simulink model "eml_hdl_design_patterns"  (R2026a)
settings: Solver=FixedStepDiscrete  StopTime=10
InitFcn:
  | errMsg  = ['\n\nThis model is only for demonstration purposes.\n\nPlease do not Simulate or code generate directly from this model. \n\nBefore generating code from this model please do copy the relevant blocks of interest from this model to a new model, place them in a subsystem, build a valid test bench around them.\n\nPlease refer to the example model ''eml_hdl_incrementer'' or HDLCoder documentation'];
  | error(sprintf(errMsg));
undefined symbols (not defined in the file or in its folder): C, gain_val, init_val, lower_limit, maxWordLength, thresh, upper_limit
libraries: simulink x2
(part 4 of 5)

== matlab function eml_hdl_design_patterns/Combinatorics/hierarchical_mimoparts/consts ==
  settings: sampleTime=1
  settings: fimath=|
      | fimath(...
      |     'RoundMode', 'floor',...
      |     'OverflowMode', 'wrap',...
      |     'ProductMode', 'SpecifyPrecision', ...
      |     'ProductWordLength', 32,...
      |     'ProductFractionLength', 20,...
      |     'SumMode', 'SpecifyPrecision', ...
      |     'SumWordLength', 32,...
      |     'SumFractionLength', 20,...
      |     'CastBeforeSum', true)
  data: const00 output; const01 output; const02 output; const03 output; const04 output; const05 output; const06 output; const07 output; const08 output; const09 output; const10 output; const11 output; const12 output; const13 output; const14 output; const15 output
function [const00, const01, const02, const03, ...
          const04, const05, const06, const07, ...
          const08, const09, const10, const11, ...
          const12, const13, const14, const15] = fcn

const00 = getfi([-1 -1 -1 -1], 1, 16, 10);
const01 = getfi([-1 -1 -1  1], 1, 16, 10);
const02 = getfi([-1 -1  1 -1], 1, 16, 10);
const03 = getfi([-1 -1  1  1], 1, 16, 10);

const04 = getfi([-1  1 -1 -1], 1, 16, 10);
const05 = getfi([-1  1 -1  1], 1, 16, 10);
const06 = getfi([-1  1  1 -1], 1, 16, 10);
const07 = getfi([-1  1  1  1], 1, 16, 10);

const08 = getfi([ 1 -1 -1 -1], 1, 16, 10);
const09 = getfi([ 1 -1 -1  1], 1, 16, 10);
const10 = getfi([ 1 -1  1 -1], 1, 16, 10);
const11 = getfi([ 1 -1  1  1], 1, 16, 10);

const12 = getfi([ 1 1 -1 -1], 1, 16, 10);
const13 = getfi([ 1 1 -1  1], 1, 16, 10);
const14 = getfi([ 1 1  1 -1], 1, 16, 10);
const15 = getfi([ 1 1  1  1], 1, 16, 10);

end

function myfi = getfi(input, issigned, wlen, flen)

fm = fimath(...
    'RoundMode', 'floor',...
    'OverflowMode', 'wrap',...
    'ProductMode', 'SpecifyPrecision', ...
    'ProductWordLength', 32,...
    'ProductFractionLength', 20,...
    'SumMode', 'SpecifyPrecision', ...
    'SumWordLength', 32,...
    'SumFractionLength', 20,...    
    'CastBeforeSum', true);

myfi = fi(input, issigned, wlen, flen, 'fimath', fm);

end

== matlab function eml_hdl_design_patterns/Combinatorics/hierarchical_mimoparts/distance ==
  settings: sampleTime=1
  settings: fimath=|
      | fimath(...
      |     'RoundMode', 'floor',...
      |     'OverflowMode', 'wrap',...
      |     'ProductMode', 'SpecifyPrecision', ...
      |     'ProductWordLength', 32,...
      |     'ProductFractionLength', 20,...
      |     'SumMode', 'SpecifyPrecision', ...
      |     'SumWordLength', 32,...
      |     'SumFractionLength', 20,...
      |     'CastBeforeSum', true)
  data: mpy00 input; mpy01 input; mpy02 input; mpy03 input; mpy04 input; mpy05 input; mpy06 input; mpy07 input; mpy08 input; mpy09 input; mpy10 input; mpy11 input; mpy12 input; mpy13 input; mpy14 input; mpy15 input; y_nums input fixdt(1,32,20) size=[1 4]; vec output
function vec = fcn(mpy00, mpy01, mpy02, mpy03, ...
          mpy04, mpy05, mpy06, mpy07, ...
          mpy08, mpy09, mpy10, mpy11, ...
          mpy12, mpy13, mpy14, mpy15, y_nums)

dout00 = distance(y_nums, mpy00);
dout01 = distance(y_nums, mpy01);
dout02 = distance(y_nums, mpy02);
dout03 = distance(y_nums, mpy03);

dout04 = distance(y_nums, mpy04);
dout05 = distance(y_nums, mpy05);
dout06 = distance(y_nums, mpy06);
dout07 = distance(y_nums, mpy07);

dout08 = distance(y_nums, mpy08);
dout09 = distance(y_nums, mpy09);
dout10 = distance(y_nums, mpy10);
dout11 = distance(y_nums, mpy11);

dout12 = distance(y_nums, mpy12);
dout13 = distance(y_nums, mpy13);
dout14 = distance(y_nums, mpy14);
dout15 = distance(y_nums, mpy15);

vec = [dout00, dout01, dout02, dout03, ...
               dout04, dout05, dout06, dout07, ...
               dout08, dout09, dout10, dout11, ...
               dout12, dout13, dout14, dout15];
           
end


function dout = distance(in1, in2)

sub_t1 = getfi(in1-in2, 1, 32, 20);
abs_t2 = getfi(abs(sub_t1), 1, 32, 20);
soe_t3 = getfi(sum(abs_t2), 1, 32, 20);

dout = soe_t3;

end




function myfi = getfi(input, issigned, wlen, flen)

fm = fimath(...
    'RoundMode', 'floor',...
    'OverflowMode', 'wrap',...
    'ProductMode', 'SpecifyPrecision', ...
    'ProductWordLength', 32,...
    'ProductFractionLength', 20,...
    'SumMode', 'SpecifyPrecision', ...
    'SumWordLength', 32,...
    'SumFractionLength', 20,...    
    'CastBeforeSum', true);

myfi = fi(input, issigned, wlen, flen, 'fimath', fm);

end

== matlab function eml_hdl_design_patterns/Combinatorics/hierarchical_mimoparts/multiply ==
  settings: sampleTime=1
  settings: fimath=|
      | fimath(...
      |     'RoundMode', 'floor',...
      |     'OverflowMode', 'wrap',...
      |     'ProductMode', 'SpecifyPrecision', ...
      |     'ProductWordLength', 32,...
      |     'ProductFractionLength', 20,...
      |     'SumMode', 'SpecifyPrecision', ...
      |     'SumWordLength', 32,...
      |     'SumFractionLength', 20,...
      |     'CastBeforeSum', true)
  data: const00 input; const01 input; const02 input; const03 input; const04 input; const05 input; const06 input; const07 input; const08 input; const09 input; const10 input; const11 input; const12 input; const13 input; const14 input; const15 input; mpy00 output; channel_matrix input fixdt(1,16,10) size=16; mpy01 output; mpy02 output; mpy03 output; mpy04 output; mpy05 output; mpy06 output; mpy07 output; mpy08 output; mpy09 output; mpy10 output; mpy11 output; mpy12 output; mpy13 output; mpy14 output; mpy15 output
function  [mpy00, mpy01, mpy02, mpy03, ...
          mpy04, mpy05, mpy06, mpy07, ...
          mpy08, mpy09, mpy10, mpy11, ...
          mpy12, mpy13, mpy14, mpy15] ...
          = fcn (const00, const01, const02, const03, ...
          const04, const05, const06, const07, ...
          const08, const09, const10, const11, ...
          const12, const13, const14, const15, ...
          channel_matrix)

mpy00 = matrix_product(const00, channel_matrix);
mpy01 = matrix_product(const01, channel_matrix);
mpy02 = matrix_product(const02, channel_matrix);
mpy03 = matrix_product(const03, channel_matrix);
  
mpy04 = matrix_product(const04, channel_matrix);
mpy05 = matrix_product(const05, channel_matrix);
mpy06 = matrix_product(const06, channel_matrix);
mpy07 = matrix_product(const07, channel_matrix);
  
mpy08 = matrix_product(const08, channel_matrix);
mpy09 = matrix_product(const09, channel_matrix);
mpy10 = matrix_product(const10, channel_matrix);
mpy11 = matrix_product(const11, channel_matrix);
  
mpy12 = matrix_product(const12, channel_matrix);
mpy13 = matrix_product(const13, channel_matrix);
mpy14 = matrix_product(const14, channel_matrix);
mpy15 = matrix_product(const15, channel_matrix);

end

function out = matrix_product(in1, in2)

const = in1';

sel1 = in2(1:4);
sel2 = in2(5:8);
sel3 = in2(9:12);
sel4 = in2(13:16);

mpy1 = get_mpy_fi(sel1 .* const, 1, 32, 20);
mpy2 = get_mpy_fi(sel2 .* const, 1, 32, 20);
mpy3 = get_mpy_fi(sel3 .* const, 1, 32, 20);
mpy4 = get_mpy_fi(sel4 .* const, 1, 32, 20);

soe1 = get_sum_fi(sum(mpy1), 1, 32, 20);
soe2 = get_sum_fi(sum(mpy2), 1, 32, 20);
soe3 = get_sum_fi(sum(mpy3), 1, 32, 20);
soe4 = get_sum_fi(sum(mpy4), 1, 32, 20);

out = [soe1, soe2, soe3, soe4];
end



function myfi = get_mpy_fi(input, issigned, wlen, flen)
% round to zero
fm = fimath(...
    'RoundMode', 'fix',... 
    'OverflowMode', 'wrap',...
    'ProductMode', 'SpecifyPrecision', ...
    'ProductWordLength', 32,...
    'ProductFractionLength', 20,...
    'SumMode', 'SpecifyPrecision', ...
    'SumWordLength', 32,...
    'SumFractionLength', 20,...    
    'CastBeforeSum', true);

myfi = fi(input, issigned, wlen, flen, 'fimath', fm);

end



function myfi = get_sum_fi(input, issigned, wlen, flen)
% drop round bits
fm = fimath(...
    'RoundMode', 'floor',... 
    'OverflowMode', 'wrap',...
    'ProductMode', 'SpecifyPrecision', ...
    'ProductWordLength', 32,...
    'ProductFractionLength', 20,...
    'SumMode', 'SpecifyPrecision', ...
    'SumWordLength', 32,...
    'SumFractionLength', 20,...    
    'CastBeforeSum', true);

myfi = fi(input, issigned, wlen, flen, 'fimath', fm);

end

== matlab function eml_hdl_design_patterns/Adders/signed_adder ==
  settings: fimath=|
      | fimath(...
      | 'RoundMode', 'floor',...
      | 'OverflowMode', 'wrap',...
      | 'ProductMode', 'FullPrecision', 'ProductWordLength', 32,...
      | 'SumMode', 'FullPrecision', 'SumWordLength', 32,...
      | 'CastBeforeSum', true)
  data: a input fixdt(1,3,0); sum output; b input fixdt(1,3,0)
function sum  = fcn(a, b)

% check default fimath settings on the block
% that define the following addition semantics

sum = a + b;

== matlab function eml_hdl_design_patterns/Combinatorics/hierarchical_mimoparts/tree_min ==
  settings: sampleTime=1
  settings: fimath=|
      | fimath(...
      |     'RoundMode', 'floor',...
      |     'OverflowMode', 'wrap',...
      |     'ProductMode', 'SpecifyPrecision', ...
      |     'ProductWordLength', 32,...
      |     'ProductFractionLength', 20,...
      |     'SumMode', 'SpecifyPrecision', ...
      |     'SumWordLength', 32,...
      |     'SumFractionLength', 20,...
      |     'CastBeforeSum', true)
  data: inVec input fixdt(1,32,20) size=[1 16]; idx output
function idx   = fcn(inVec)
%--------------------------------------------------------------------------
% Tree implementation min function for vector input of length 64
%--------------------------------------------------------------------------
[minimum, idx] = tree_min(inVec);
            
end

function [minval, idx] = tree_min(invec)

% initialize outputs

% first level of comparison
inidx = uint8(1:16);
[lvlonemin, lvloneidx] = vector_min(invec, inidx);

% second level of comparison
[lvltwomin, lvltwoidx] = vector_min(lvlonemin, lvloneidx);

% third level of comparison
[lvlthreemin, lvlthreeidx] = vector_min(lvltwomin, lvltwoidx);

% final comparison
[minval, idx] = vector_min(lvlthreemin, lvlthreeidx);

end

% Minimum subfuction for tree implementation
function [minvec, idxvec] = vector_min(invec, inidx)
    
lengthminvec = uint8(length(invec)/2);
%lengthminvec = uint8(bitshift(invec, -1));
minvec = getfi(zeros(lengthminvec, 1), 1, 12, 6);
idxvec = uint8(zeros(lengthminvec, 1));

for i=1:lengthminvec
    % get two consecutive values
    idx2 = int8(i)+int8(i); %i*2
    idx1 = int8(idx2) - int8(1); %i*2-1
    % get elements
    val1 = invec(idx1);
    val2 = invec(idx2);
    % compare them and select minimum
    if le(val1, val2)
        minvec(i) = val1;
        idxvec(i) = inidx(idx1);
    else
        minvec(i) = val2;
        idxvec(i) = inidx(idx2);
    end
end

end


function myfi = getfi(input, issigned, wlen, flen)

fm = fimath(...
    'RoundMode', 'floor',... 
    'OverflowMode', 'wrap',...
    'ProductMode', 'SpecifyPrecision', ...
    'ProductWordLength', 32,...
    'ProductFractionLength', 20,...
    'SumMode', 'SpecifyPrecision', ...
    'SumWordLength', 32,...
    'SumFractionLength', 20,...    
    'CastBeforeSum', true);

myfi = fi(input, issigned, wlen, flen, 'fimath', fm);

end

== matlab function eml_hdl_design_patterns/Combinatorics/monolithic_mimoparts ==
  settings: fimath=|
      | fimath(...
      |     'RoundMode', 'floor',...
      |     'OverflowMode', 'wrap',...
      |     'ProductMode', 'SpecifyPrecision', ...
      |     'ProductWordLength', 32,...
      |     'ProductFractionLength', 20,...
      |     'SumMode', 'SpecifyPrecision', ...
      |     'SumWordLength', 32,...
      |     'SumFractionLength', 20,...
      |     'CastBeforeSum', true)
  data: y_nums input fixdt(1,32,20) size=[1 4]; idx output; channel_matrix input fixdt(1,16,10) size=16
function idx = fcn(y_nums, channel_matrix)

% This function illustrates some of the key pieces of a MIMO decoder, but
% is meant only for educational value at this time.
% 
% Key MATLAB code features used in this example:
% 
% 1. Creating vector constants
% 2. Using 'SpecifyPrecision' option in fimath
% 3. Indexing of vector operands
% 4. Transpose operations
% 5. Elementwise product operations
% 6. Sum of elements operation using sum input
% 7. Tree min function implementation
% 8. Vector ports
%

const00 = getfi([-1 -1 -1 -1], 1, 16, 10);
const01 = getfi([-1 -1 -1  1], 1, 16, 10);
const02 = getfi([-1 -1  1 -1], 1, 16, 10);
const03 = getfi([-1 -1  1  1], 1, 16, 10);

const04 = getfi([-1  1 -1 -1], 1, 16, 10);
const05 = getfi([-1  1 -1  1], 1, 16, 10);
const06 = getfi([-1  1  1 -1], 1, 16, 10);
const07 = getfi([-1  1  1  1], 1, 16, 10);

const08 = getfi([ 1 -1 -1 -1], 1, 16, 10);
const09 = getfi([ 1 -1 -1  1], 1, 16, 10);
const10 = getfi([ 1 -1  1 -1], 1, 16, 10);
const11 = getfi([ 1 -1  1  1], 1, 16, 10);

const12 = getfi([ 1 1 -1 -1], 1, 16, 10);
const13 = getfi([ 1 1 -1  1], 1, 16, 10);
const14 = getfi([ 1 1  1 -1], 1, 16, 10);
const15 = getfi([ 1 1  1  1], 1, 16, 10);

mpy00 = matrix_product(const00, channel_matrix);
mpy01 = matrix_product(const01, channel_matrix);
mpy02 = matrix_product(const02, channel_matrix);
mpy03 = matrix_product(const03, channel_matrix);
  
mpy04 = matrix_product(const04, channel_matrix);
mpy05 = matrix_product(const05, channel_matrix);
mpy06 = matrix_product(const06, channel_matrix);
mpy07 = matrix_product(const07, channel_matrix);
  
mpy08 = matrix_product(const08, channel_matrix);
mpy09 = matrix_product(const09, channel_matrix);
mpy10 = matrix_product(const10, channel_matrix);
mpy11 = matrix_product(const11, channel_matrix);
  
mpy12 = matrix_product(const12, channel_matrix);
mpy13 = matrix_product(const13, channel_matrix);
mpy14 = matrix_product(const14, channel_matrix);
mpy15 = matrix_product(const15, channel_matrix);

dout00 = distance(y_nums, mpy00);
dout01 = distance(y_nums, mpy01);
dout02 = distance(y_nums, mpy02);
dout03 = distance(y_nums, mpy03);

dout04 = distance(y_nums, mpy04);
dout05 = distance(y_nums, mpy05);
dout06 = distance(y_nums, mpy06);
dout07 = distance(y_nums, mpy07);

dout08 = distance(y_nums, mpy08);
dout09 = distance(y_nums, mpy09);
dout10 = distance(y_nums, mpy10);
dout11 = distance(y_nums, mpy11);

dout12 = distance(y_nums, mpy12);
dout13 = distance(y_nums, mpy13);
dout14 = distance(y_nums, mpy14);
dout15 = distance(y_nums, mpy15);

idx = TreeMin([dout00, dout01, dout02, dout03, ...
               dout04, dout05, dout06, dout07, ...
               dout08, dout09, dout10, dout11, ...
               dout12, dout13, dout14, dout15]);
           
end

function out = matrix_product(in1, in2)

sel1 = in2(1:4);
sel2 = in2(5:8);
sel3 = in2(9:12);
sel4 = in2(13:16);

% mpy1 = getfi(sel1*in1, 1, 32, 20);
% mpy2 = getfi(sel2*in1, 1, 32, 20);
% mpy3 = getfi(sel3*in1, 1, 32, 20);
% mpy4 = getfi(sel4*in1, 1, 32, 20);

mpy1 = getfi(sel1 .* in1', 1, 32, 20);
mpy2 = getfi(sel2 .* in1', 1, 32, 20);
mpy3 = getfi(sel3 .* in1', 1, 32, 20);
mpy4 = getfi(sel4 .* in1', 1, 32, 20);

soe1 = getfi(sum(mpy1), 1, 32, 20);
soe2 = getfi(sum(mpy2), 1, 32, 20);
soe3 = getfi(sum(mpy3), 1, 32, 20);
soe4 = getfi(sum(mpy4), 1, 32, 20);

out = [soe1, soe2, soe3, soe4];

end


function dout = distance(in1, in2)

sub_t1 = getfi(in1-in2, 1, 32, 20);
abs_t2 = getfi(abs(sub_t1), 1, 32, 20);
soe_t3 = getfi(sum(abs_t2), 1, 32, 20);

dout = soe_t3;

end


function [idx, minimum]  = TreeMin(nsm)
%--------------------------------------------------------------------------
% Tree implementation min function for vector input of length 64
%--------------------------------------------------------------------------
[minimum, idx] = tree_min(nsm);
            
end

function [minval, idx] = tree_min(invec)

% initialize outputs
% minval = getfi(0, 1, 12, 6);
% idx = 0;

% first level of comparison
inidx = uint8(1:16);
[lvlonemin, lvloneidx] = vector_min(invec, inidx);

% second level of comparison
[lvltwomin, lvltwoidx] = vector_min(lvlonemin, lvloneidx);

% third level of comparison
[lvlthreemin, lvlthreeidx] = vector_min(lvltwomin, lvltwoidx);

% final comparison
[minval, idx] = vector_min(lvlthreemin, lvlthreeidx);


end

% Minimum subfuction for tree implementation
function [minvec, idxvec] = vector_min(invec, inidx)
    
lengthminvec = length(invec)/2;
%lengthminvec = uint8(bitshift(invec, -1));
minvec = getfi(zeros(lengthminvec, 1), 1, 12, 6);
idxvec = uint8(zeros(lengthminvec, 1));

for i=1:lengthminvec
    % get two consecutive values
    idx2 = int8(i)+int8(i); %i*2
    idx1 = int8(idx2) - int8(1); %i*2-1
    % get elements
    val1 = invec(idx1);
    val2 = invec(idx2);
    % compare them and select minimum
    if le(val1, val2)
        minvec(i) = val1;
        idxvec(i) = inidx(idx1);
    else
        minvec(i) = val2;
        idxvec(i) = inidx(idx2);
    end
end

end


function myfi = getfi(input, issigned, wlen, flen)

fm = fimath(...
    'RoundMode', 'floor',... 
    'OverflowMode', 'wrap',...
    'ProductMode', 'SpecifyPrecision', ...
    'ProductWordLength', 32,...
    'ProductFractionLength', 20,...
    'SumMode', 'SpecifyPrecision', ...
    'SumWordLength', 32,...
    'SumFractionLength', 20,...    
    'CastBeforeSum', true);

myfi = fi(input, issigned, wlen, flen, 'fimath', fm);

end

== matlab function eml_hdl_design_patterns/Complex/Complex Integer Delay ==
  settings: fimath=|
      | fimath(...
      | 'RoundMode', 'floor',...
      | 'OverflowMode', 'wrap',...
      | 'ProductMode', 'FullPrecision', 'ProductWordLength', 32,...
      | 'SumMode', 'FullPrecision', 'SumWordLength', 32,...
      | 'CastBeforeSum', true)
  data: u input; y output
function y = fcn(u)

% The Integer Delay block delays its input by N sample periods. 
% The block accepts one input and generates one output, both of which
% can be scalar or vector. If the input is a vector, all elements of the 
% vector are delayed by the same sample period.

% In this example N is hardwired as 4; This function behaves as Integer 
% delay block and delays inputs by 4 sample hits.

persistent u_d;
if isempty(u_d)
    u_d = fi(complex(zeros(1,4)), numerictype(u), fimath(u));
end

y = u_d(4);

u_d = [u, u_d(1), u_d(2), u_d(3)];

== matlab function eml_hdl_design_patterns/Register Files/dualport_regfile ==
  settings: fimath=|
      | fimath(...
      | 'RoundMode', 'floor',...
      | 'OverflowMode', 'wrap',...
      | 'ProductMode', 'FullPrecision', 'ProductWordLength', 32,...
      | 'SumMode', 'FullPrecision', 'SumWordLength', 32,...
      | 'CastBeforeSum', true)
  data: writedata input int8; readdata output; writeaddr input uint8; written input boolean; readaddr input uint8
function readdata = fcn(writedata, writeaddr, written, readaddr)

% Synchronous register file in eML

% this generates a "register-file" and 
% does not help infer a true RAM in synthesis

% nonetheless, they are very useful for simulation and 
% can be replaced at synthesis time with code that 
% does infer a RAM or a black-box RAM.


persistent reg_file;
if isempty(reg_file)
    reg_file = fi(zeros(1, 64), 0, 8, 0);
end

trf = reg_file;
trf(writeaddr) = writedata;

% decide new reg file based on written flag
if (written)
    new_rf = trf;
else
    new_rf = reg_file;
end

% read data
readdata = reg_file(readaddr);

% update reg file
reg_file = new_rf;

== matlab function eml_hdl_design_patterns/Register Files/triport_regfile ==
  settings: fimath=|
      | fimath(...
      | 'RoundMode', 'floor',...
      | 'OverflowMode', 'wrap',...
      | 'ProductMode', 'FullPrecision', 'ProductWordLength', 32,...
      | 'SumMode', 'FullPrecision', 'SumWordLength', 32,...
      | 'CastBeforeSum', true)
  data: writedata input int8; readdata_a output; writeaddr input uint8; written input boolean; readaddr_a input uint8; readaddr_b input uint8; readdata_b output
function [readdata_a, readdata_b]= fcn(writedata, writeaddr, written, readaddr_a, readaddr_b)

% Synchronous Dual Port register file in eML

% this generates a "register-file" and 
% does not help infer a true RAM in synthesis
% Nonetheless, they are very useful for simulation and 
% can be replaced at synthesis time with code that 
% does infer a RAM or a black-box RAM.


persistent reg_file;
if isempty(reg_file)
    reg_file = fi(zeros(1, 64), 0, 8, 0);
end

trf = reg_file;
trf(writeaddr) = writedata;

% decide new reg file based on written flag
if (written)
    new_rf = trf;
else
    new_rf = reg_file;
end

% read data portA
readdata_a = reg_file(readaddr_a);

% read data portB
readdata_b = reg_file(readaddr_b);

% update reg file
reg_file = new_rf;

== matlab function eml_hdl_design_patterns/ShiftAdd Algs/cordic/InitValues/Init ==
  settings: fimath=|
      | fimath(...
      | 'RoundMode', 'floor',...
      | 'OverflowMode', 'wrap',...
      | 'ProductMode', 'FullPrecision', 'ProductWordLength', 32,...
      | 'SumMode', 'FullPrecision', 'SumWordLength', 32,...
      | 'CastBeforeSum', true)
  data: x0 output fixdt(1,24,8); y0 output fixdt(1,24,8); h_mode output boolean; r0 output fixdt(1,24,8); rot_mode output uint8; lut_values output fixdt(1,16,8) size=[1 8]; p_or_rate output uint8; cordic_gain output fixdt(1,24,23); angle_gain output fixdt(1,24,22)
function [x0, y0, ...    
    h_mode,...
    r0, rot_mode, ...    
    lut_values, ...
    p_or_rate, ...
    cordic_gain, ...
    angle_gain] = INIT

% from mask input
p_or_rate = uint8(8);

x0 = getfi(1); 
y0 = getfi(0);

r0 = getfi(0);

% hyperbolic mode
h_mode = false;

% rotation mode
rot_mode = uint8(2); 

%cg = 1/get_cordic_gain(8, 'Circular');
%cordic_gain = fi(cg, 1, 24, 23);
cordic_gain = fi(0.607259154319763, 1, 24, 23);

angle_gain = fi(1, 1, 24, 22);

%sincos_val = (atan([1, 1/2, 1/4, 1/8, 1/16, 1/32, 1/64, 1/128]))*180/pi;
%lut_values = fi(sincos_val, 1, 16, 8);

lut_values = fi([45, 26.56640625, 14.03515625, 7.125, 3.578125, 1.7890625, 0.89453125, 0.44921875], 1, 16, 8);


function fival = getfi(val)

nt = numerictype(1, 24, 8);

fm = fimath(...
    'RoundMode', 'floor',...
    'OverflowMode', 'wrap',...
    'ProductMode', 'FullPrecision', 'ProductWordLength', 32,...
    'SumMode', 'FullPrecision', 'SumWordLength', 32,...
    'CastBeforeSum', true);

fival = fi(val, nt, fm);

== matlab function eml_hdl_design_patterns/ShiftAdd Algs/cordic/cordic_core/Q Correction ==
  settings: fimath=|
      | fimath(...
      | 'RoundMode', 'floor',...
      | 'OverflowMode', 'wrap',...
      | 'ProductMode', 'FullPrecision', 'ProductWordLength', 32,...
      | 'SumMode', 'FullPrecision', 'SumWordLength', 32,...
      | 'CastBeforeSum', true)
  data: theta input fixdt(1,24,8); left_quad output; angle output
function [left_quad, angle] = Q_Correction(theta)

angle = theta;
left_quad = angle <= 270 && angle >= 90;

if left_quad
    angle = getfi(angle - getfi(180));
end


function fival = getfi(val)

nt = numerictype(1, 24, 8);

fm = fimath(...
    'RoundMode', 'floor',...
    'OverflowMode', 'wrap',...
    'ProductMode', 'FullPrecision', 'ProductWordLength', 32,...
    'SumMode', 'FullPrecision', 'SumWordLength', 32,...
    'CastBeforeSum', true);

fival = fi(val, nt, fm);

== matlab function eml_hdl_design_patterns/Counters/gray_counter ==
  settings: sampleTime=.1
  settings: fimath=|
      | fimath(...
      | 'RoundMode', 'floor',...
      | 'OverflowMode', 'wrap',...
      | 'ProductMode', 'FullPrecision', 'ProductWordLength', 32,...
      | 'SumMode', 'FullPrecision', 'SumWordLength', 32,...
      | 'CastBeforeSum', true)
  data: clear input boolean; count output fixdt(0,4,0) size=1
function count = fcn(clear)

% A gray counter is a binary counter with the following conversion logic:

% 1. the first gray bit (msb) is same as first binary bit
% 2. the second gray bit is determined by xoring the second binary with the first binary bit and so on;
%    that is each pair of adjacent bits are xor'ed to get the next gray bit.
%
% This counter is configured to rollover.  Set result_fm to 'saturate'
% if roll over is not desirable.

result_nt = numerictype(0,4,0);
result_fm = fimath('OverflowMode', 'wrap', 'RoundMode', 'floor');

persistent bin_count;
if isempty(bin_count)
    bin_count = fi(0, result_nt, result_fm);
end

persistent gray_count;
if isempty(gray_count)
    gray_count = fi(0, result_nt, result_fm); %#ok<NASGU>
end

count = gray_count;

if clear
    bin_count =  fi(0, result_nt, result_fm);
    gray_count =  fi(0, result_nt, result_fm);
else
    inc = bin_count + fi(1, result_nt, result_fm);
    bin_count = fi(inc, result_nt, result_fm);

    gray_count = bitshift(bin_count, -1);
    gray_count = bitxor( gray_count, bin_count );
end

== matlab function eml_hdl_design_patterns/Complex/Complex Tap Delay ==
  settings: fimath=|
      | fimath(...
      | 'RoundMode', 'floor',...
      | 'OverflowMode', 'wrap',...
      | 'ProductMode', 'FullPrecision', 'ProductWordLength', 32,...
      | 'SumMode', 'FullPrecision', 'SumWordLength', 32,...
      | 'CastBeforeSum', true)
  data: u input; d1 output; d2 output; d3 output; d4 output
function [d1, d2, d3, d4] = fcn(u)
%The Tapped Delay function delays its input by the specified number 
% of sample periods, and outputs all the delayed versions.

% In this example N is hardwired to 4.

persistent u_d;
if isempty(u_d)
    u_d = fi(complex(zeros(1,4)), numerictype(u), fimath(u));
end

d1 = u_d(1);
d2 = u_d(2);
d3 = u_d(3);
d4 = u_d(4);

u_d = [u_d(1), u_d(2), u_d(3), u];

== matlab function eml_hdl_design_patterns/Word Twiddlers/signal_distance ==
  settings: fimath=|
      | fimath(...
      | 'RoundMode', 'floor',...
      | 'OverflowMode', 'wrap',...
      | 'ProductMode', 'FullPrecision', 'ProductWordLength', 32,...
      | 'SumMode', 'FullPrecision', 'SumWordLength', 32,...
      | 'CastBeforeSum', true)
  data: u input fixdt(0,5,0); y output; v input fixdt(0,5,0)
function y = fcn(u, v)

% get all bits of u
t1 = bitget(u, int8(5:-1:1));

% get all bits of v in reverse order
t2 = bitget(v, int8(1:1:5));

% xor the bits
t3 = xor(t1, t2);

% find number of bits that are equal to 1

t = uint8(t3);
y = uint8(0);
for i=uint8(1:5)
    y = y+t(i);
end

== matlab function eml_hdl_design_patterns/ShiftAdd Algs/cordic/cordic_core/controller ==
  settings: updateMethod=DISCRETE  sampleTime=1/8
  settings: fimath=|
      | fimath(...
      | 'RoundMode', 'floor',...
      | 'OverflowMode', 'wrap',...
      | 'ProductMode', 'FullPrecision', 'ProductWordLength', 32,...
      | 'SumMode', 'FullPrecision', 'SumWordLength', 32,...
      | 'CastBeforeSum', true)
  data: ctrl output; address output; d_valid output; rate input
function [ctrl,address,d_valid] = controller(rate)

persistent count;
if isempty(count)
    count = uint8(1);
end

% output address
address = count;

% update count value
count = get_en_ctr_val(rate);

% send control signals based on current count value
ctrl = (count == 1);
d_valid = (count == 8);



function count = get_en_ctr_val(rate)

persistent count_val;
if isempty(count_val)
    count_val = uint8(1);
end

% output count
count = count_val;

% update count
if count >= rate
    next_cnt_val = uint8(1);
else
    next_cnt_val = uint8(count+1);
end


count_val = uint8(next_cnt_val);

== matlab function eml_hdl_design_patterns/ShiftAdd Algs/cordic/cordic_core/cordic_rotator/get_sign ==
  settings: fimath=|
      | fimath(...
      | 'RoundMode', 'floor',...
      | 'OverflowMode', 'wrap',...
      | 'ProductMode', 'FullPrecision', 'ProductWordLength', 32,...
      | 'SumMode', 'FullPrecision', 'SumWordLength', 32,...
      | 'CastBeforeSum', true)
  data: y input; x input; z input; r0 input; sign output boolean; r_mode input
function sign = get_sign(y, x, z, r0, r_mode)

sign = false;

switch (r_mode)
    case 0
        sign = x <= r0;
    case 1
        sign = y  <= r0;
    case 2
        sign = z >= r0;
end

== matlab function eml_hdl_design_patterns/ShiftAdd Algs/cordic/cordic_core/cordic_rotator/x_comp ==
  settings: fimath=|
      | fimath(...
      | 'RoundMode', 'floor',...
      | 'OverflowMode', 'wrap',...
      | 'ProductMode', 'FullPrecision', 'ProductWordLength', 32,...
      | 'SumMode', 'FullPrecision', 'SumWordLength', 32,...
      | 'CastBeforeSum', true)
  data: y input fixdt(1,24,8) size=1; next_x output fixdt(1,24,8) size=1; x0 input fixdt(1,24,8) size=1; h_mode input boolean size=1; ctrl input boolean size=1; addr input uint8 size=1; sign input boolean; store_x output fixdt(1,24,8); reg_x input fixdt(1,24,8)
function [next_x, store_x]   = x_comp(y, x0, h_mode, ctrl, addr, sign, reg_x)

y = bitshift(y, -int8(addr-1));

if h_mode    
    new_sign = sign;
else
    new_sign = ~sign;
end

next_x = z_accumulator(new_sign, reg_x, y);

% update delay line
if (ctrl)
    store_x = x0;
else
    store_x = next_x;
end


function acc = z_accumulator(add, x, y)

if (add)
    acc = getfi(x+y);
else
    acc = getfi(x-y);
end


function fival = getfi(val)

nt = numerictype(1, 24, 8);
fm = fimath(...
    'RoundMode', 'floor',...
    'OverflowMode', 'wrap',...
    'ProductMode', 'FullPrecision', 'ProductWordLength', 32,...
    'SumMode', 'FullPrecision', 'SumWordLength', 32,...
    'CastBeforeSum', true);

fival = fi(val, nt, fm);

== matlab function eml_hdl_design_patterns/ShiftAdd Algs/cordic/cordic_core/cordic_rotator/y_comp ==
  settings: fimath=|
      | fimath(...
      | 'RoundMode', 'floor',...
      | 'OverflowMode', 'wrap',...
      | 'ProductMode', 'FullPrecision', 'ProductWordLength', 32,...
      | 'SumMode', 'FullPrecision', 'SumWordLength', 32,...
      | 'CastBeforeSum', true)
  data: next_y output fixdt(1,24,8); x input fixdt(1,24,8); y0 input fixdt(1,24,8); ctrl input boolean; addr input uint8; sign input boolean; store_y output fixdt(1,24,8); reg_y input fixdt(1,24,8)
function [next_y, store_y]  = y_comp(x, y0, ctrl, addr, sign, reg_y)

x = bitshift(x, -int8(addr-1));

next_y = z_accumulator(sign, x, reg_y);

if (ctrl)
    store_y = y0;
else
    store_y = next_y;
end


function acc = z_accumulator(add, x, y)

if (add)
    acc = getfi(y+x);
else
    acc = getfi(y-x);
end

function fival = getfi(val)

nt = numerictype(1, 24, 8);

fm = fimath(...
    'RoundMode', 'floor',...
    'OverflowMode', 'wrap',...
    'ProductMode', 'FullPrecision', 'ProductWordLength', 32,...
    'SumMode', 'FullPrecision', 'SumWordLength', 32,...
    'CastBeforeSum', true);

fival = fi(val, nt, fm);

== matlab function eml_hdl_design_patterns/FSMs/mealy_fsm ==
  settings: fimath=|
      | fimath(...
      | 'RoundMode', 'nearest',...
      | 'OverflowMode', 'saturate',...
      | 'ProductMode', 'FullPrecision', 'ProductWordLength', 128,...
      | 'SumMode', 'FullPrecision', 'SumWordLength', 128,...
      | 'CastBeforeSum', true)
  data: A input boolean; Z output boolean size=1
function Z = fcn(A)

persistent mealy_state_reg;
if isempty(mealy_state_reg)
    mealy_state_reg = fi(0, 0, 2, 0);   
end

S1 = 0;
S2 = 1;
S3 = 2;
S4 = 3;

switch (mealy_state_reg) 
    
    case S1
        
        if (A)
            Z = true;
            mealy_state_reg(1) = S1;
        else
            Z = false;            
            mealy_state_reg(1) = S2;
        end
        
    case S2
        
        if (A)
            Z = false;
            mealy_state_reg(1) = S1;
        else
            Z = true;
            mealy_state_reg(1) = S2;
        end
        
    case S3
        

        if (A)
            Z = false;            
            mealy_state_reg(1) = S2;
        else
            Z = true;            
            mealy_state_reg(1) = S3;
        end
        
    case S4
        

        if (A)
            Z = true;
            mealy_state_reg(1) = S1;
        else
            Z = false;            
            mealy_state_reg(1) = S3;
        end        
        
    otherwise
        
        Z = false;
end

== matlab function eml_hdl_design_patterns/ShiftAdd Algs/cordic/cordic_core/cordic_rotator/z_comp ==
  settings: fimath=|
      | fimath(...
      | 'RoundMode', 'floor',...
      | 'OverflowMode', 'wrap',...
      | 'ProductMode', 'FullPrecision', 'ProductWordLength', 32,...
      | 'SumMode', 'FullPrecision', 'SumWordLength', 32,...
      | 'CastBeforeSum', true)
  data: next_z output fixdt(1,24,8); z0 input fixdt(1,24,8); lut_values input fixdt(1,16,8) size=[1 8]; ctrl input boolean; addr input uint8; sign input boolean; reg_z input fixdt(1,24,8); store_z output
function [next_z, store_z]   = z_comp(z0, lut_values, ctrl, addr, sign, reg_z)

y = lut_values(addr);

%sign = ~sign;
next_z = z_accumulator(~sign, reg_z, y);

% update delay line
if (ctrl)
    store_z = z0;
else
    store_z = next_z;
end

function acc = z_accumulator(add, x, y)

if (add)
    acc = getfi(x+y);
else
    acc = getfi(x-y);
end


function fival = getfi(val)

nt = numerictype(1, 24, 8);

fm = fimath(...
    'RoundMode', 'floor',...
    'OverflowMode', 'wrap',...
    'ProductMode', 'FullPrecision', 'ProductWordLength', 32,...
    'SumMode', 'FullPrecision', 'SumWordLength', 32,...
    'CastBeforeSum', true);

fival = fi(val, nt, fm);

== matlab function eml_hdl_design_patterns/ShiftAdd Algs/cordic/gain_correction ==
  settings: updateMethod=DISCRETE  sampleTime=1/8
  settings: fimath=|
      | fimath(...
      | 'RoundMode', 'floor',...
      | 'OverflowMode', 'wrap',...
      | 'ProductMode', 'SpecifyPrecision', 'ProductWordLength', 32,...
      | 'SumMode', 'SpecifyPrecision', 'SumWordLength', 32,...
      | 'CastBeforeSum', true)
  data: sine output fixdt(1,24,8); cosine output fixdt(1,24,8); xn input fixdt(1,24,8); yn input fixdt(1,24,8); zn input fixdt(1,24,8); q_correction input boolean; enable input boolean; cordic_gain input fixdt(1,24,23); angle_gain input fixdt(1,24,22); new_angle output fixdt(1,24,8)
function [sine, cosine, new_angle] = gain_correction(xn, yn, zn, q_correction, enable, cordic_gain, angle_gain)

persistent x_reg;
if isempty(x_reg)
    x_reg = getfi(0);
end

persistent y_reg;
if isempty(y_reg)
    y_reg = getfi(0);
end

persistent z_reg;
if isempty(z_reg)
    z_reg = getfi(0);
end

xg = getfi(cordic_gain*xn);
yg = getfi(cordic_gain*yn);

[xout, yout] = vector_correction(xg, yg, cordic_gain, q_correction);
zout = z_correction(zn, q_correction, angle_gain);

sine = x_reg;
cosine = y_reg;
new_angle = z_reg;

if (enable)
    x_reg = xout;
    y_reg = yout;
    z_reg = zout;
end

function [xout, yout] = vector_correction(x, y, c0, q_correction)

if q_correction
    direction = getfi(-1);
else
    direction = getfi(1);
end

xout = getfi(x*direction);
yout = getfi(y*direction);


function z_c = z_correction(zn, z_corr, z_gain)

t1 = getfi(zn);
t2 = getfi(uint8(z_corr));
zadd = getfi(t1+t2);

z_c = getfi(zadd * z_gain);



function fival = getfi(val)

nt = numerictype(1, 24, 8);

fm = fimath(...
    'RoundMode', 'floor',...
    'OverflowMode', 'wrap',...
    'ProductMode', 'SpecifyPrecision', 'ProductWordLength', 32,...
    'SumMode', 'SpecifyPrecision', 'SumWordLength', 32,...
    'CastBeforeSum', true);

fival = fi(val, nt, fm);

== matlab function eml_hdl_design_patterns/Complex/Complex Tap Delay Vector ==
  settings: fimath=|
      | fimath(...
      | 'RoundMode', 'floor',...
      | 'OverflowMode', 'wrap',...
      | 'ProductMode', 'FullPrecision', 'ProductWordLength', 32,...
      | 'SumMode', 'FullPrecision', 'SumWordLength', 32,...
      | 'CastBeforeSum', true)
  data: u input; y output
function y = fcn(u)
% The Tapped Delay function delays its input by the specified number 
% of sample periods, and outputs all the delayed versions in a vector
% form.

% In this example N is hardwired to 4.

persistent u_d;
if isempty(u_d)
    u_d = fi(complex(zeros(1,4)), numerictype(u), fimath(u));
end

y = u_d;

u_d = [u, u_d(1), u_d(2), u_d(3)];

== matlab function eml_hdl_design_patterns/DSP Ops/dsp_fold ==
  settings: fimath=|
      | fimath(...
      | 'RoundMode', 'floor',...
      | 'OverflowMode', 'wrap',...
      | 'ProductMode', 'FullPrecision', 'ProductWordLength', 32,...
      | 'SumMode', 'FullPrecision', 'SumWordLength', 32,...
      | 'CastBeforeSum', true)
  data: x input fixdt(0,5,2) size=[1 10]; y output; n input uint8 size=[1 10]; n1 output
function [y, n1] = fcn(x, n)

% each sample of x(n) is flipped around n==0
%   y(n) = x(-n);

y = fliplr(x);
n1 = -fliplr(n);

== matlab function eml_hdl_design_patterns/DSP Ops/dsp_scale ==
  settings: fimath=|
      | fimath(...
      | 'RoundMode', 'floor',...
      | 'OverflowMode', 'wrap',...
      | 'ProductMode', 'FullPrecision', 'ProductWordLength', 32,...
      | 'SumMode', 'FullPrecision', 'SumWordLength', 32,...
      | 'CastBeforeSum', true)
  data: x input fixdt(0,5,2); y output; alpha input fixdt(0,4,1)
function y  = fcn(x, alpha)

y = alpha * x;

== matlab function eml_hdl_design_patterns/DSP Ops/dsp_shift ==
  settings: fimath=|
      | fimath(...
      | 'RoundMode', 'floor',...
      | 'OverflowMode', 'wrap',...
      | 'ProductMode', 'FullPrecision', 'ProductWordLength', 32,...
      | 'SumMode', 'FullPrecision', 'SumWordLength', 32,...
      | 'CastBeforeSum', true)
  data: x input fixdt(0,5,2); y output; m input uint8; k input uint8; n output
function [y, n] = fcn(x, m, k)

% during signal shift each sample of x(n) is shifted by an amount k
% to obtain a shifted sequence y(n)
%  	y(n) = x(n-k)
% let m = n-k then n = m+k and the above operation is given by
% 	y(m+k) = x(m)
% hence the shift operation has no effect on vector x, but the 
% position vector is changed by adding k to each element.

n = m+k;
y = x;

== matlab function eml_hdl_design_patterns/DSP Ops/dsp_sum ==
  settings: fimath=|
      | fimath(...
      | 'RoundMode', 'floor',...
      | 'OverflowMode', 'wrap',...
      | 'ProductMode', 'FullPrecision', 'ProductWordLength', 32,...
      | 'SumMode', 'FullPrecision', 'SumWordLength', 32,...
      | 'CastBeforeSum', true)
  data: x input fixdt(0,5,2) size=[1 10]; y output
function y  = fcn(x)

% x is a signal of type ufix5_En2 and length [1 x 10]

n1 = 1;
n2 = 10;

y = sum(x(n1:n2));

== matlab function eml_hdl_design_patterns/Parity Generators/xor_parity_blk ==
  settings: fimath=|
      | fimath(...
      | 'RoundMode', 'floor',...
      | 'OverflowMode', 'wrap',...
      | 'ProductMode', 'FullPrecision', 'ProductWordLength', 32,...
      | 'SumMode', 'FullPrecision', 'SumWordLength', 32,...
      | 'CastBeforeSum', true)
  data: a input fixdt(0,4,0); result output; b input fixdt(0,4,0); c input fixdt(0,4,0); d input fixdt(0,4,0)
function result  = fcn(a, b, c, d)

t1 = bitxor(a,b);
t2 = bitxor(c,d);
result = bitxor(t1, t2);

== matlab function eml_hdl_design_patterns/Misc/agc ==
  settings: fimath=|
      | fimath(...
      | 'RoundMode', 'floor',...
      | 'OverflowMode', 'wrap',...
      | 'ProductMode', 'FullPrecision', 'ProductWordLength', 32,...
      | 'SumMode', 'FullPrecision', 'SumWordLength', 32,...
      | 'CastBeforeSum', true)
  data: real_in input fixdt(1,10,9); real_out output; imag_in input fixdt(1,10,9); imag_out output; gain_out output
function [real_out, imag_out, gain_out] = fcn(real_in, imag_in)

% Automatic Gain Controller

% The ability to set the gain level in a circuit and have it 
% control itself is a very useful function.
%
% An example use of AGC would be to control the gain so the signals for 
% a digital downconverter (DDC) and digital upconverter (DUC) 
% would be in a specific range so the A/D that processes 
% the IF of the mixers does not get over-driven by the amplitude 
% of the input signals

% compute magnitude
mag_out = mag_approx(real_in, imag_in);

% quantize it
qmag_out = fi(mag_out, 0, 10, 10, fimath(mag_out));
cic_out = cic_filter(qmag_out);

% updated gain
nt = numerictype(0, 6, 6);
fm = fimath(cic_out);

c1 = fi(1/16, nt, fm);
gain_out = fi(c1 * cic_out, nt, fm);

% adjust gain
c1 = fi(0.5, nt, fm);
tsub = fi(c1 - gain_out, nt, fm);

persistent g_integrator
if isempty(g_integrator)
    g_integrator = fi(0, nt, fm);
end

% compute final integrator output
tadd = fi(tsub + g_integrator, nt, fm);

g_integrator = tadd;

% compute outputs
real_out = g_integrator * real_in;
imag_out = g_integrator * imag_in;
gain_out = g_integrator;

end

% magnitude approximation
function approx_mag_out = mag_approx(real_in, imag_in)

ar_in = abs(real_in);
ai_in = abs(imag_in);

iq_max = max(ar_in, ai_in);
iq_min = min(ar_in, ai_in);

approx_mag_out = iq_max + iq_min * fi(0.4, numerictype(iq_min), fimath(iq_max));

end

% cic filter
function cic_out = cic_filter(cic_in)

nt = numerictype(cic_in);
fm = fimath(cic_in);

persistent cicdiff;
if isempty(cicdiff)
    cicdiff = fi(zeros(1, 16), nt, fm);
end

% find cicdiff
tsub = fi(cic_in - cicdiff(1), nt, fm);

% update delay line
cicdiff = [cicdiff(2:16), cic_in];

persistent cichold;
if isempty(cichold)
    cichold = fi(0, nt, fm);
end

persistent cicintegrator;
if isempty(cicintegrator)
    cicintegrator = fi(0, nt, fm);
end

% update output with previous value of integrator
cic_out = cicintegrator;

% compute new value into integrator
tadd = fi(cichold + cicintegrator, nt, fm);

% update hold and integrator delay lines
cichold = tsub;
cicintegrator = tadd;

end

== matlab function eml_hdl_design_patterns/Sorters/bubble_sort ==
  settings: fimath=|
      | fimath(...
      | 'RoundMode', 'floor',...
      | 'OverflowMode', 'wrap',...
      | 'ProductMode', 'FullPrecision', 'ProductWordLength', 32,...
      | 'SumMode', 'FullPrecision', 'SumWordLength', 32,...
      | 'CastBeforeSum', true)
  data: u input uint8 size=[1 8]; y output
function y = fcn(u)

% this function implements a bubble sort algorithm

for i = 1:length(u)
    for j = 1:length(u) - 1
        if u(j) > u(j+1)
            tmp = u(j+1);
            u(j+1) = u(j);
            u(j) = tmp;
        end
    end
end

y = u;

== matlab function eml_hdl_design_patterns/Sorters/bitonic_sort ==
  settings: fimath=|
      | fimath(...
      | 'RoundMode', 'floor',...
      | 'OverflowMode', 'wrap',...
      | 'ProductMode', 'FullPrecision', 'ProductWordLength', 32,...
      | 'SumMode', 'FullPrecision', 'SumWordLength', 32,...
      | 'CastBeforeSum', true)
  data: inVec input uint8 size=[1 8]; outVec output
function outVec = fcn(inVec)

% this function implements bitonicsort algorithm

outVec = bitonicSort8( inVec );

end

function out = bitonicSort8( in )
    out = fi( zeros(8, 1), 0, 8, 0 );
    
    out(1:4) = bitonicSort4(in(1:4), true);
    out(5:8) = bitonicSort4( in(5:8), false );
    out = bitonicMerge8( out, true );
end

function out = bitonicSort4( in, direction )
    out = fi( zeros(4, 1), 0, 8, 0 );
    out(1:2) = bitonicSort2( in(1:2), true);
    out(3:4) = bitonicSort2( in(3:4), false );
    out = bitonicMerge4( out, direction );
end

function out = bitonicSort2( in, direction )
  out = bitonicMerge2( in, direction );
end

function out = bitonicMerge8( in, direction )
    out = fi( zeros(8, 1), 0, 8, 0 );
    for i = 1:4
        tmp = compare( [in(i); in(i + 4)], direction );
        out(i) = tmp(1);
        out(i+4) = tmp(2);
    end
    out(1:4) = bitonicMerge4( out(1:4), direction );
    out(5:8) = bitonicMerge4( out(5:8), direction );
end

function out = bitonicMerge4( in, direction )
    out = fi( zeros(4, 1), 0, 8, 0 );
    for i = 1:2
        tmp = compare( [in(i); in(i + 2)], direction );
        out(i) = tmp(1);
        out(i+2) = tmp(2);
    end
    out(1:2) = bitonicMerge2( out(1:2), direction );
    out(3:4) = bitonicMerge2( out(3:4), direction );
end

function out = bitonicMerge2( in, direction)
    out = compare( [in(1); in(2)], direction );
end

function out = compare( in, direction )
   if direction == (in(1) > in(2) )
       out = [in(2); in(1)];
   else
       out = in;
   end
end

== matlab function eml_hdl_design_patterns/Misc/gcd ==
  settings: fimath=|
      | fimath(...
      | 'RoundMode', 'nearest',...
      | 'OverflowMode', 'saturate',...
      | 'ProductMode', 'FullPrecision', 'ProductWordLength', 128,...
      | 'SumMode', 'FullPrecision', 'SumWordLength', 128,...
      | 'CastBeforeSum', true)
  data: gcd_out output; x_in input int16; rfd output size=1; ready output; y_in input int16; go input boolean
function [gcd_out, rfd, ready] = fcn(x_in, y_in, go)

% This function block impelemnts the gcd algorithm shipping 
% in hdlcodergcd.mdl in eML

persistent gcd_state_reg;
if isempty(gcd_state_reg)
    gcd_state_reg = uint8(0);
end

persistent x_reg;
if isempty(x_reg)
    x_reg = int16(0);
end

persistent y_reg;
if isempty(y_reg)
    y_reg = int16(0);
end

Init = uint8(0);
Idle = uint8(1);
S1 = uint8(2);
S2 = uint8(3);
S3 = uint8(4);
S4 = uint8(5);
S5 = uint8(6);

x = x_reg;
y = y_reg;

gcd_out = y;

switch uint8(gcd_state_reg)

    case Init
        x_reg = x;
        y_reg = y;
        rfd = true;
        ready = false;
        gcd_state_reg = Idle;

    case Idle

        if go
            x_reg = x_in;
            y_reg = y_in;
            rfd = false;
            ready = false;
            gcd_state_reg = S1;
            
        else
            x_reg = x;
            y_reg = y;
            rfd = true;
            ready = false;
            gcd_state_reg = Idle;
        end

    case S1
        x_reg = x;
        y_reg = y;
        rfd = false;
        ready = false;
        gcd_state_reg = S2;

    case S2

        if x > y
            x_reg = x - y;
            y_reg = y;
            rfd = false;
            ready = false;
            gcd_state_reg = S3;
            
        elseif x < y
            x_reg = x;
            y_reg = y - x;
            rfd = false;
            ready = false;
            gcd_state_reg = S4;
            
        else
            x_reg = x;
            y_reg = y;
            rfd = false;
            ready = true;
            gcd_state_reg = S5;
        end

    case S3
        x_reg = x;
        y_reg = y;
        rfd = false;
        ready = false;
        gcd_state_reg = S2;

    case S4
        x_reg = x;
        y_reg = y;
        rfd = false;
        ready = false;
        gcd_state_reg = S2;

    case S5
        x_reg = x;
        y_reg = y;
        rfd = true;
        ready = false;
        gcd_state_reg = Idle;

    otherwise
        x_reg = x;
        y_reg = y;
        rfd = true;
        ready = false;
        gcd_state_reg = Idle;

end

== matlab function eml_hdl_design_patterns/Misc/dot_product ==
  settings: fimath=|
      | fimath(...
      | 'RoundMode', 'floor',...
      | 'OverflowMode', 'wrap',...
      | 'ProductMode', 'FullPrecision', ...
      | 'SumMode', 'FullPrecision', ...
      | 'CastBeforeSum', true)
  data: A input int16; S output int16; B input int16
function S  = fcn(A, B) 

S = int16(sum(A .* B));

== matlab function eml_hdl_design_patterns/Complex/Complex Unit Delay ==
  settings: fimath=|
      | fimath(...
      | 'RoundMode', 'floor',...
      | 'OverflowMode', 'wrap',...
      | 'ProductMode', 'FullPrecision', 'ProductWordLength', 32,...
      | 'SumMode', 'FullPrecision', 'SumWordLength', 32,...
      | 'CastBeforeSum', true)
  data: u input; y output
function y = fcn(u)
% Complex unit delay

% The Unit Delay block delays its input by the specified sample period.
% The block accepts one input and generates one output, which can
% be either both scalar or both vector. If the input is a vector, 
% all elements of the vector are delayed by the same sample period.
%
% You specify the block output for the first sampling period with the 
% Initial value to the persistent variable.
%

% y is same as u delayed by one sample period.

% output of this block at the first sample hit is decided by the initial 
% value of this persistent variable.
persistent u_d;
if isempty(u_d)
    u_d = fi(complex(-1), numerictype(u), fimath(u));
end

% return delayed input from last sample time hit
y = u_d;

% store the current input to be used later
u_d = u;

== matlab function eml_hdl_design_patterns/Misc/bit_vector_shuffle ==
  settings: fimath=|
      | fimath(...
      | 'RoundMode', 'floor',...
      | 'OverflowMode', 'wrap',...
      | 'ProductMode', 'FullPrecision', 'ProductWordLength', 32,...
      | 'SumMode', 'FullPrecision', 'SumWordLength', 32,...
      | 'CastBeforeSum', true)
  data: u2 input fixdt(0,4,0); y output; u1 input fixdt(0,4,0)
function y = fcn(u2, u1)

% this block shows how to quickly do rewiring of input input words

y = [bitsliceget(u1,1,1) bitsliceget(u2,1,1) bitsliceget(u1,2,2) bitsliceget(u2, 2,2) bitsliceget(u1,3,3) bitsliceget(u2,3,3) bitsliceget(u1,4,4) bitsliceget(u2,4,4)];
